simulink model "2026-09-17_fourier_npu_algorithm"  (R2026a)
settings: Solver=FixedStepDiscrete  StopTime=0  FixedStep=1
undefined symbols (not defined in the file or in its folder): VIB_INPUT

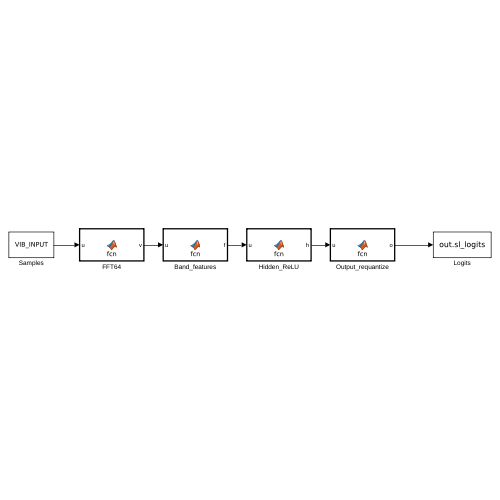
[thumbnail: Simulink's stored preview of the top-level diagram]
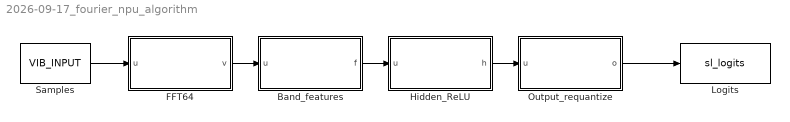
== system 2026-09-17_fourier_npu_algorithm ==
  Band_features : MATLAB Function  TreatAsAtomicUnit=on
  FFT64 : MATLAB Function  TreatAsAtomicUnit=on
  Hidden_ReLU : MATLAB Function  TreatAsAtomicUnit=on
  Logits : ToWorkspace  VariableName=sl_logits  SampleTime=-1
  Output_requantize : MATLAB Function  TreatAsAtomicUnit=on
  Samples : Constant  Value=VIB_INPUT
  wires:
  Samples/1 -> FFT64/1(u)
  FFT64/1(v) -> Band_features/1(u)
  Band_features/1(f) -> Hidden_ReLU/1(u)
  Hidden_ReLU/1(h) -> Output_requantize/1(u)
  Output_requantize/1(o) -> Logits/1

== matlab function 2026-09-17_fourier_npu_algorithm/FFT64 ==
  data: u input; v output
function v=fcn(u)
v=fourier_fft_sl(u);
end

== matlab function 2026-09-17_fourier_npu_algorithm/Hidden_ReLU ==
  data: u input; h output
function h=fcn(u)
w=[-50 -15 -48 -44;-48 -16 -50 -39;-67 -9 -62 -58;-61 -13 -65 -51];
b=[414;403;540;513];
h=max(0,min(127,floor((w*double(u(:))+b)/2^4)));
end

== matlab function 2026-09-17_fourier_npu_algorithm/Output_requantize ==
  data: u input; o output
function o=fcn(u)
w=[52 54 64 52;-55 -59 -58 -56];
b=[-1943;1943];
o=max(-128,min(127,floor((w*double(u(:))+b)/2^5)));
end

== matlab function 2026-09-17_fourier_npu_algorithm/Band_features ==
  data: u input; f output
function f=fcn(u)
f=fourier_features_sl(u);
end
